simulink model "t_type_lcl_sin3_demo"  (R2025b)
settings: Solver=ode23tb  StartTime=0.0  StopTime=t_stop  MaxStep=max_step  RelTol=1e-3
PreLoadFcn:
  | demo_root=fileparts(fileparts(get_param(bdroot,'FileName'))); run(fullfile(demo_root,'parameters','thesis_demo_parameters.m')); clear demo_root;
undefined symbols (not defined in the file): Cf, I_ref_pk, Kdist, Kp, Ksin3, L1, L2, Lg, R1, R2, Rd, sin3_enable, V_grid_pk, Vdc, w_grid
settings Model: Creator=bob  LastModifiedBy=bob
settings DataIOCC: SignalLogging=off

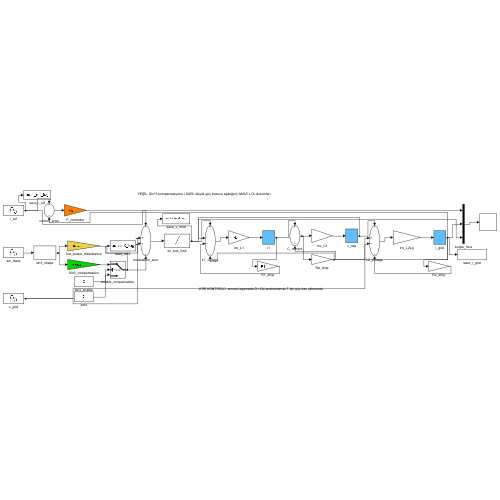
[thumbnail: Simulink's stored preview of the top-level diagram]
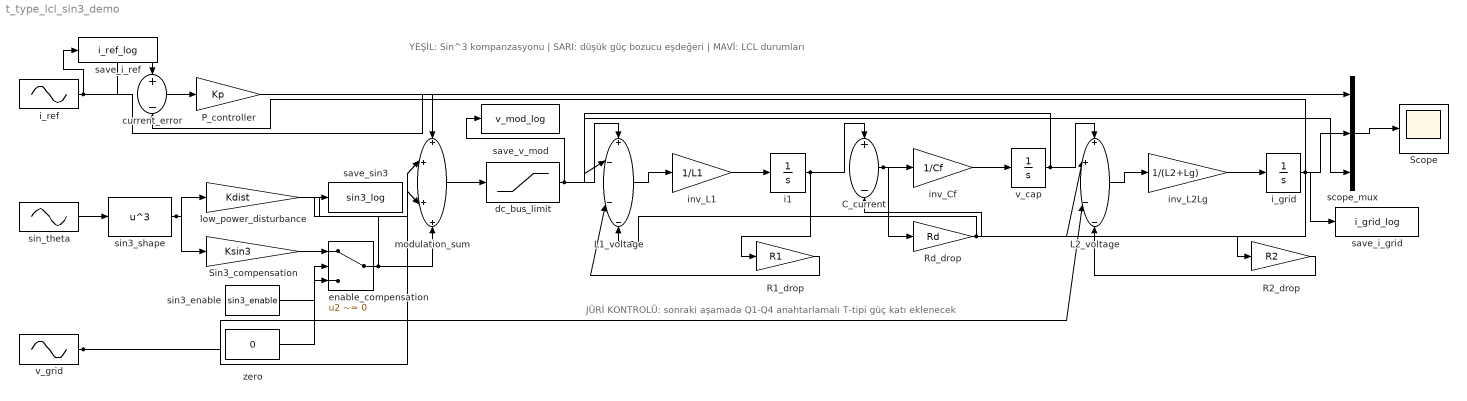
== system t_type_lcl_sin3_demo ==
  note: YEŞİL: Sin^3 kompanzasyonu | SARI: düşük güç bozucu eşdeğeri | MAVİ: LCL durumları
  note: JÜRİ KONTROLÜ: sonraki aşamada Q1-Q4 anahtarlamalı T-tipi güç katı eklenecek
  C_current : Sum  Inputs=+-
  L1_voltage : Sum  Inputs=+---
  L2_voltage : Sum  Inputs=++--
  P_controller : Gain  Gain=Kp
  R1_drop : Gain  Gain=R1
  R2_drop : Gain  Gain=R2
  Rd_drop : Gain  Gain=Rd
  Scope : Scope
  Sin3_compensation : Gain  Gain=Ksin3
  current_error : Sum  Inputs=+-
  dc_bus_limit : Saturate  UpperLimit=Vdc/2  LowerLimit=-Vdc/2
  enable_compensation : Switch  Criteria=u2 ~= 0  Threshold=0.5  SaturateOnIntegerOverflow=off  InputSameDT=off
  i1 : Integrator
  i_grid : Integrator
  i_ref : Sin  Amplitude=I_ref_pk  Frequency=w_grid  SampleTime=0
  inv_Cf : Gain  Gain=1/Cf
  inv_L1 : Gain  Gain=1/L1
  inv_L2Lg : Gain  Gain=1/(L2+Lg)
  low_power_disturbance : Gain  Gain=Kdist
  modulation_sum : Sum  Inputs=++++
  save_i_grid : ToWorkspace  VariableName=i_grid_log  SaveFormat=Timeseries  SampleTime=-1
  save_i_ref : ToWorkspace  VariableName=i_ref_log  SaveFormat=Timeseries  SampleTime=-1
  save_sin3 : ToWorkspace  VariableName=sin3_log  SaveFormat=Timeseries  SampleTime=-1
  save_v_mod : ToWorkspace  VariableName=v_mod_log  SaveFormat=Timeseries  SampleTime=-1
  scope_mux : Mux  Inputs=3
  sin3_enable : Constant  Value=sin3_enable
  sin3_shape : Fcn  Expr=u^3
  sin_theta : Sin  Frequency=w_grid  SampleTime=0
  v_cap : Integrator
  v_grid : Sin  Amplitude=V_grid_pk  Frequency=w_grid  SampleTime=0
  zero : Constant  Value=0
  wires:
  i_ref/1 -> current_error/1, save_i_ref/1, scope_mux/1
  current_error/1 -> P_controller/1
  sin_theta/1 -> sin3_shape/1
  sin3_shape/1 -> low_power_disturbance/1, Sin3_compensation/1
  Sin3_compensation/1 -> enable_compensation/1
  sin3_enable/1 -> enable_compensation/2
  zero/1 -> enable_compensation/3
  P_controller/1 -> modulation_sum/1
  v_grid/1 -> modulation_sum/2, L2_voltage/3
  low_power_disturbance/1 -> modulation_sum/3
  enable_compensation/1 -> modulation_sum/4, save_sin3/1
  modulation_sum/1 -> dc_bus_limit/1
  dc_bus_limit/1 -> L1_voltage/1, save_v_mod/1, scope_mux/3
  v_cap/1 -> L1_voltage/2, L2_voltage/1
  i1/1 -> R1_drop/1, C_current/1
  R1_drop/1 -> L1_voltage/3
  Rd_drop/1 -> L1_voltage/4, L2_voltage/2
  L1_voltage/1 -> inv_L1/1
  inv_L1/1 -> i1/1
  i_grid/1 -> C_current/2, R2_drop/1, current_error/2, save_i_grid/1, scope_mux/2
  C_current/1 -> inv_Cf/1, Rd_drop/1
  inv_Cf/1 -> v_cap/1
  R2_drop/1 -> L2_voltage/4
  L2_voltage/1 -> inv_L2Lg/1
  inv_L2Lg/1 -> i_grid/1
  scope_mux/1 -> Scope/1
